simulink model "surrogate_model_14"  (R2026a)
settings: Solver=VariableStepAuto
settings Model: Creator=shuki  LastModifiedBy=shuki

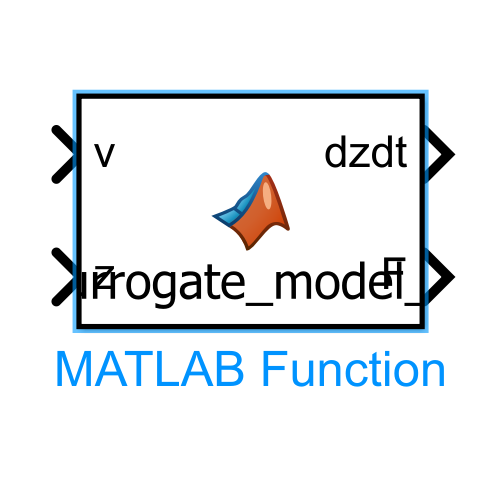
[thumbnail: Simulink's stored preview of the top-level diagram]
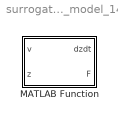
== system surrogate_model_14 ==
  MATLAB Function : MATLAB Function  TreatAsAtomicUnit=on

== matlab function surrogate_model_14/MATLAB Function ==
  data: dzdt output; F output; v input; z input
function [dzdt, F] = surrogate_model_9(v, z)

    S0 = 10^5;
    C1 = 0.85228235;
    C2 = -0.13998671;
    C3 = 6.7612834;
    C4 = 7.2667336;

    dzdt = v - z*( abs(C1*S0*v) + abs(C3 + C2*(S0^2*v*z)) - C4);

    F = 10^5 * z + 316.2277 * dzdt + 0.4 * v;

end
